simulink model "step06_model"  (R2024a)
settings: Solver=VariableStepAuto  StartTime=0.0  StopTime=10.0  RelTol=1e-3
libraries: fl_lib x14, ee_lib x5, nesl_utility x4
settings Model: Creator=Jonathan  LastModifiedBy=Jonathan
settings DebuggingCC: UnderspecifiedInitializationDetection=Classic  MergeDetectMultiDrivingBlocksExec=none
settings ModelReferenceCC: PropagateSignalLabelsOutOfModel=off

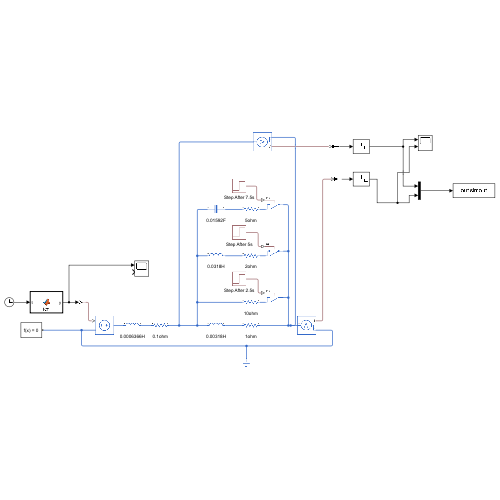
[thumbnail: Simulink's stored preview of the top-level diagram]
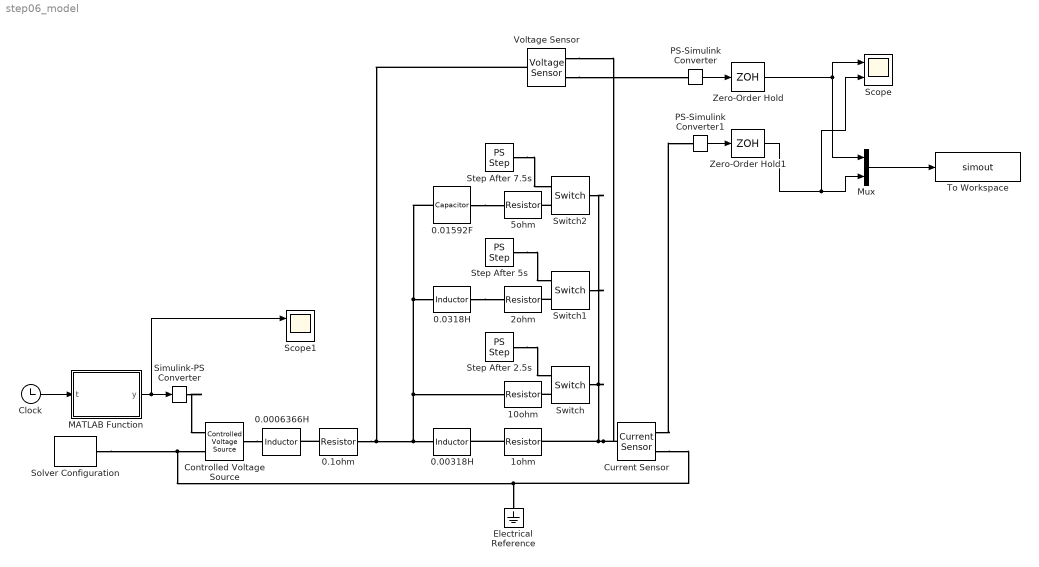
== system step06_model ==
  0.0006366H : ee_lib/Passive/Inductor  l=0.0006366 H  enable_L_tol=ee.enum.toleranceApplication.none  L_tol=20  tol_distribution=ee.enum.toleranceDistribution.uniform  nSigma=4  r=0 Ohm  g=1e-9 1/Ohm  enable_operating_limits=ee.enum.enable.no  operating_limit_action=ee.enum.passive.reportOpLim.warn  max_working_current=1 A  power_rating=1 W  enable_faults=ee.enum.enable.no  fault_action=simscape.enum.assert.action.none  lambdaPercent=50  k_faulted=0.9999  turnsShort=ee.enum.passive.inductor.turnsShortOption.no  openCct=ee.enum.enable.no  groundShort=ee.enum.passive.inductor.groundShortOption.no  groundShortG=0 1/Ohm  tau_fault=1e-3 s  fault_trigger=ee.enum.faults.faultTrigger.temporal  t_fault=1 s  max_permissible_voltage=100 V  n_fail_on_voltage=1  max_permissible_current=1 A  t_fail_on_current=1 s  i_L_specify=off  i_L_priority=High  i_L=0 A  i_L_nominal_specify=off  i_L_nominal_value=1  i_L_nominal_unit=A  faulted_specify=off  faulted_priority=None  faulted=0
  0.00318H : ee_lib/Passive/Inductor  l=0.00318 H  enable_L_tol=ee.enum.toleranceApplication.none  L_tol=20  tol_distribution=ee.enum.toleranceDistribution.uniform  nSigma=4  r=0 Ohm  g=1e-9 1/Ohm  enable_operating_limits=ee.enum.enable.no  operating_limit_action=ee.enum.passive.reportOpLim.warn  max_working_current=1 A  power_rating=1 W  enable_faults=ee.enum.enable.no  fault_action=simscape.enum.assert.action.none  lambdaPercent=50  k_faulted=0.9999  turnsShort=ee.enum.passive.inductor.turnsShortOption.no  openCct=ee.enum.enable.no  groundShort=ee.enum.passive.inductor.groundShortOption.no  groundShortG=0 1/Ohm  tau_fault=1e-3 s  fault_trigger=ee.enum.faults.faultTrigger.temporal  t_fault=1 s  max_permissible_voltage=100 V  n_fail_on_voltage=1  max_permissible_current=1 A  t_fail_on_current=1 s  i_L_specify=off  i_L_priority=High  i_L=0 A  i_L_nominal_specify=off  i_L_nominal_value=1  i_L_nominal_unit=A  faulted_specify=off  faulted_priority=None  faulted=0
  0.01592F : fl_lib/Electrical/Electrical Elements/Capacitor  c=0.01592 F  r=1e-6 Ohm  g=0 1/Ohm  i_specify=off  i_priority=None  i=0 A  i_nominal_specify=off  i_nominal_value=1  i_nominal_unit=A  v_specify=off  v_priority=None  v=0 V  v_nominal_specify=off  v_nominal_value=1  v_nominal_unit=V  vc_specify=off  vc_priority=High  vc=0 V  vc_nominal_specify=off  vc_nominal_value=1  vc_nominal_unit=V
  0.0318H : ee_lib/Passive/Inductor  l=0.0318 H  enable_L_tol=ee.enum.toleranceApplication.none  L_tol=20  tol_distribution=ee.enum.toleranceDistribution.uniform  nSigma=4  r=0 Ohm  g=1e-9 1/Ohm  enable_operating_limits=ee.enum.enable.no  operating_limit_action=ee.enum.passive.reportOpLim.warn  max_working_current=1 A  power_rating=1 W  enable_faults=ee.enum.enable.no  fault_action=simscape.enum.assert.action.none  lambdaPercent=50  k_faulted=0.9999  turnsShort=ee.enum.passive.inductor.turnsShortOption.no  openCct=ee.enum.enable.no  groundShort=ee.enum.passive.inductor.groundShortOption.no  groundShortG=0 1/Ohm  tau_fault=1e-3 s  fault_trigger=ee.enum.faults.faultTrigger.temporal  t_fault=1 s  max_permissible_voltage=100 V  n_fail_on_voltage=1  max_permissible_current=1 A  t_fail_on_current=1 s  i_L_specify=off  i_L_priority=High  i_L=0 A  i_L_nominal_specify=off  i_L_nominal_value=1  i_L_nominal_unit=A  faulted_specify=off  faulted_priority=None  faulted=0
  0.1ohm : ee_lib/Passive/Resistor  R=0.1 Ohm  enable_R_tol=ee.enum.toleranceApplication.none  R_tol=5  tol_distribution=ee.enum.toleranceDistribution.uniform  nSigma=4  enable_operating_limits=ee.enum.enable.no  operating_limit_action=ee.enum.passive.reportOpLim.warn  power_rating=1 W  max_working_voltage=100 V  enable_faults=ee.enum.enable.no  fault_action=simscape.enum.assert.action.none  R_faulted=inf Ohm  fault_trigger=ee.enum.faults.faultTrigger.temporal  t_fault=1 s  max_permissible_current=1 A  t_fail_on_current=1 s  noise_mode=ee.enum.sources.noise.Disabled  Tdevice=25 degC  sample_time=1e-3 s  repeatability=ee.enum.ic.repeatability.notRepeatable  user_seed=0  auto_seed=3499211588  faulted_specify=off  faulted_priority=None  faulted=0  power_derating_T1=70 degC  power_derating_T2=155 degC  operating_temperature_range_vec=[-50, 150] degC  alpha=3.93e-3 1/K  Tmeas=25 degC  thermal_mass=100 J/K  temperature_specify=off  temperature_priority=High  temperature=298.15 K  temperature_nominal_specify=off  temperature_nominal_value=1  temperature_nominal_unit=K
  10ohm : fl_lib/Electrical/Electrical Elements/Resistor  R=10 Ohm  i_specify=off  i_priority=None  i=0 A  i_nominal_specify=off  i_nominal_value=1  i_nominal_unit=A  v_specify=off  v_priority=None  v=0 V  v_nominal_specify=off  v_nominal_value=1  v_nominal_unit=V
  1ohm : ee_lib/Passive/Resistor  R=1 Ohm  enable_R_tol=ee.enum.toleranceApplication.none  R_tol=5  tol_distribution=ee.enum.toleranceDistribution.uniform  nSigma=4  enable_operating_limits=ee.enum.enable.no  operating_limit_action=ee.enum.passive.reportOpLim.warn  power_rating=1 W  max_working_voltage=100 V  enable_faults=ee.enum.enable.no  fault_action=simscape.enum.assert.action.none  R_faulted=inf Ohm  fault_trigger=ee.enum.faults.faultTrigger.temporal  t_fault=1 s  max_permissible_current=1 A  t_fail_on_current=1 s  noise_mode=ee.enum.sources.noise.Disabled  Tdevice=25 degC  sample_time=1e-3 s  repeatability=ee.enum.ic.repeatability.notRepeatable  user_seed=0  auto_seed=3890346746  faulted_specify=off  faulted_priority=None  faulted=0  power_derating_T1=70 degC  power_derating_T2=155 degC  operating_temperature_range_vec=[-50, 150] degC  alpha=3.93e-3 1/K  Tmeas=25 degC  thermal_mass=100 J/K  temperature_specify=off  temperature_priority=High  temperature=298.15 K  temperature_nominal_specify=off  temperature_nominal_value=1  temperature_nominal_unit=K
  2ohm : fl_lib/Electrical/Electrical Elements/Resistor  R=2 Ohm  i_specify=off  i_priority=None  i=0 A  i_nominal_specify=off  i_nominal_value=1  i_nominal_unit=A  v_specify=off  v_priority=None  v=0 V  v_nominal_specify=off  v_nominal_value=1  v_nominal_unit=V
  5ohm : fl_lib/Electrical/Electrical Elements/Resistor  R=5 Ohm  i_specify=off  i_priority=None  i=0 A  i_nominal_specify=off  i_nominal_value=1  i_nominal_unit=A  v_specify=off  v_priority=None  v=0 V  v_nominal_specify=off  v_nominal_value=1  v_nominal_unit=V
  Clock : Clock
  Controlled Voltage Source : fl_lib/Electrical/Electrical Sources/Controlled Voltage Source
  Current Sensor : fl_lib/Electrical/Electrical Sensors/Current Sensor
  Electrical Reference : fl_lib/Electrical/Electrical Elements/Electrical Reference
  MATLAB Function : MATLAB Function  TreatAsAtomicUnit=on
  Mux : Mux  Inputs=2
  PS-Simulink Converter : nesl_utility/PS-Simulink Converter  PhysicalDomain=network_engine_domain  SubClassName=ps_output  LeftPortType=input  RightPortType=output  PseudoPeriodic=off  Frequencies=[]  VectorFormat=inherit  Unit=inherit  AffineConversion=off
  PS-Simulink Converter1 : nesl_utility/PS-Simulink Converter  PhysicalDomain=network_engine_domain  SubClassName=ps_output  LeftPortType=input  RightPortType=output  PseudoPeriodic=off  Frequencies=[]  VectorFormat=inherit  Unit=inherit  AffineConversion=off
  Scope : Scope  NumInputPorts=2
  Scope1 : Scope  NumInputPorts=2
  Simulink-PS Converter : nesl_utility/Simulink-PS Converter  PhysicalDomain=network_engine_domain  SubClassName=ps_input  LeftPortType=input  RightPortType=output  PseudoPeriodic=off  Frequencies=[]  NoiseDistribution=none  NoiseParameters=[]  Unit=1  AffineConversion=off  FilteringAndDerivatives=provide  SimscapeFilterOrder=1  InputFilterTimeConstant=0.001  UdotUserProvided=0
  Solver Configuration : nesl_utility/Solver Configuration  PhysicalDomain=network_engine_domain  SubClassName=solver  LeftPortType=input  RightPortType=generic  Tones=[]  Harmonics=[]  SimulateNoise=off  Profile=off  UseLocalSampling=off  EnableSwitchedLinearOptims=on  FrequencyDomain=off  UseCCode=off  RelTol=0.001  AbsTol=0.001  MinStep=1e-09  ToWorkspace=off  RevertToSquareIcSolve=off  NumHomotopyIterations=100  PhasorMode=off  PhasorModeNumHarmonics=1  ConsistencySolver=NEWTON_XTOL_AFTER_FTOL  IndexReductionMethod=DerivativeReplacement  DoDC=off  ResidualTolerance=1e-09  ConsistencyTolSource=GLOBAL  ConsistencyAbsTol=0.001  ConsistencyRelTol=0.001  ConsistencyTolFactor=0.001  UseLocalSolver=off  LocalSolverChoice=NE_BACKWARD_EULER_ADVANCER  ResolveIndetEquations=on  FunctionEvalNumThread=1  LocalSolverSampleTime=0.001  DoFixedCost=off  MaxNonlinIter=3  MaxModeIter=2  ComputeImpulses=off  ImpulseIterations=2  LinearAlgebra=auto  LinearAlgebraNumThread=0  EquationFormulation=NE_TIME_EF  DelaysMemoryBudget=1024  AutomaticFiltering=on  FilteringTimeConstant=0.001  PartitionStorageMethod=AS_NEEDED  PartitionMemoryBudget=1024  PartitionMethod=ROBUST  MultibodyUseLocalSolver=off  MultibodyLocalSolverChoice=ODE1  MultibodyLocalSolverSampleTime=0.001
  Step After 2.5s : fl_lib/Physical Signals/Sources/PS Step  step_time=2.5 s  initial_value=0  final_value=1
  Step After 5s : fl_lib/Physical Signals/Sources/PS Step  step_time=5 s  initial_value=0  final_value=1
  Step After 7.5s : fl_lib/Physical Signals/Sources/PS Step  step_time=7.5 s  initial_value=0  final_value=1
  Switch : fl_lib/Electrical/Electrical Elements/Switch  R_closed=0.01 Ohm  G_open=1e-8 1/Ohm  Threshold=0.5  i_specify=off  i_priority=None  i=0 A  i_nominal_specify=off  i_nominal_value=1  i_nominal_unit=A  v_specify=off  v_priority=None  v=0 V  v_nominal_specify=off  v_nominal_value=1  v_nominal_unit=V
  Switch1 : fl_lib/Electrical/Electrical Elements/Switch  R_closed=0.01 Ohm  G_open=1e-8 1/Ohm  Threshold=0.5  i_specify=off  i_priority=None  i=0 A  i_nominal_specify=off  i_nominal_value=1  i_nominal_unit=A  v_specify=off  v_priority=None  v=0 V  v_nominal_specify=off  v_nominal_value=1  v_nominal_unit=V
  Switch2 : fl_lib/Electrical/Electrical Elements/Switch  R_closed=0.01 Ohm  G_open=1e-8 1/Ohm  Threshold=0.5  i_specify=off  i_priority=None  i=0 A  i_nominal_specify=off  i_nominal_value=1  i_nominal_unit=A  v_specify=off  v_priority=None  v=0 V  v_nominal_specify=off  v_nominal_value=1  v_nominal_unit=V
  To Workspace : ToWorkspace  VariableName=simout  SaveFormat=Timeseries  SampleTime=1/8192
      settings: MaxDataPoints=81920
  Voltage Sensor : fl_lib/Electrical/Electrical Sensors/Voltage Sensor
  Zero-Order Hold : ZeroOrderHold  SampleTime=1/10000
  Zero-Order Hold1 : ZeroOrderHold  SampleTime=1/10000
  wires:
  PS-Simulink Converter/1 -> Zero-Order Hold/1
  Zero-Order Hold/1 -> Scope/1, Mux/1
  Zero-Order Hold1/1 -> Mux/2, Scope/2
  PS-Simulink Converter1/1 -> Zero-Order Hold1/1
  Mux/1 -> To Workspace/1
  Clock/1 -> MATLAB Function/1(t)
  MATLAB Function/1(y) -> Scope1/1, Simulink-PS Converter/1
  connections:
  1ohm/LConn1 -- 0.00318H/RConn1
  Solver Configuration/RConn1 -- Controlled Voltage Source/RConn2 -- Current Sensor/RConn2 -- Electrical Reference/LConn1
  Voltage Sensor/RConn1 -- PS-Simulink Converter/LConn1
  0.1ohm/RConn1 -- 0.00318H/LConn1 -- 0.01592F/LConn1 -- 0.0318H/LConn1 -- 10ohm/LConn1 -- Voltage Sensor/LConn1
  Current Sensor/LConn1 -- Voltage Sensor/RConn2 -- Switch2/LConn1 -- Switch1/LConn1 -- Switch/LConn1 -- 1ohm/RConn1
  Current Sensor/RConn1 -- PS-Simulink Converter1/LConn1
  0.1ohm/LConn1 -- 0.0006366H/RConn1
  Controlled Voltage Source/LConn1 -- 0.0006366H/LConn1
  Switch/RConn2 -- 10ohm/RConn1
  Step After 2.5s/RConn1 -- Switch/RConn1
  Step After 5s/RConn1 -- Switch1/RConn1
  Switch1/RConn2 -- 2ohm/RConn1
  Step After 7.5s/RConn1 -- Switch2/RConn1
  Switch2/RConn2 -- 5ohm/RConn1
  0.01592F/RConn1 -- 5ohm/LConn1
  0.0318H/RConn1 -- 2ohm/LConn1
  Simulink-PS Converter/RConn1 -- Controlled Voltage Source/RConn1

== matlab function step06_model/MATLAB Function ==
  data: t input; y output
function y = fcn(t)

    % MATLAB Function Block: Generates 230V RMS (325.27V peak) sine wave
    % with linear frequency modulation between 48 Hz and 52 Hz over 10 seconds.
    
    A = 230 * sqrt(2);

    if t <= 10
        % Instantaneous frequency f(t) = 48 + 0.4*t
        % Phase phi = 2 * pi * integral(f(t) dt) = 2 * pi * (48*t + 0.2*t^2)
        phi = 2 * pi * (48 * t + 0.2 * t^2);
    else
        % Fixed frequency at 52 Hz after 10 seconds with continuous phase
        phi = 2 * pi * (52 * t - 20);
    end
    
    y = A * sin(phi);

    %y = 230 * sqrt(2)*sin(2*pi()*50*t);
end
